simulink model "PMSM_Simulink"  (R2024b)
settings: Solver=FixedStepDiscrete  StartTime=0.0  StopTime=10  FixedStep=0.0000625/200  RelTol=1e-3
libraries: simulink x12, slpidlib x3, spsDCVoltageSourceLib x1, spsPermanentMagnetSynchronousMachineLib x1, spsUniversalBridgeLib x1, sps_lib x1
(part 2 of 2)

== stateflow chart PMSM_Simulink/PMSM_MC1/MC_LowFrqTask /MotModeCtr/Chart ==
  state Calibrate
    state Init
      en:
      MotCtrMode = 0;
    state Calibrate1
      en:
      MotCtrMode=1;
      MotCalThetae=1.046;//60°
    state Calibrate2
      en:
      MotOffsetBuff[0]=Ecode_Cnt-166;
      MotCtrMode=2;
      MotCalThetae=2.093;//120°
    state RngChk
      en:
      MotOffsetBuff[1]=Ecode_Cnt-333;
      RangeCheck();
    (default) -> Init
    Init -> Calibrate1 : [MotorSpdRef !=0]
    Calibrate1 -> Calibrate2 : [after(1.5,sec )]
    Calibrate2 -> RngChk : [after(1.5,sec )]
  state RangeCheck [function]
    (default) -> (junction 31)
    (junction 31) -> (junction 33) [order 1] : [abs(MotOffsetBuff[0]-MotOffsetBuff[1])>1000]
    (junction 33) -> (junction 36) : {
        | MotCalNormal=0;
        | }
    (junction 31) -> (junction 35) [order 2] : {
        | MotCalNormal=1;
        | MotOffset=(MotOffsetBuff[0]+MotOffsetBuff[1]/2)
        | }
    (junction 36) -> (junction 35)
    (junction 35) -> (junction 42)
  state Normal
    state Stop
      en:
      MotCtrMode=4;
    state Run
      en:
      MotCtrMode=5;
    (default) -> Stop
    Run -> Stop : [MotorSpdRef==0]
    Stop -> Run : [MotorSpdRef!=0]
  state CallFailed
    en:
    MotCtrMode=3;
  (default) -> Calibrate
  CallFailed -> Calibrate : [MotorSpdRef==0]
  RngChk -> CallFailed [order 1] : [MotCalNormal==0]
  RngChk -> Normal [order 2] : [MotCalNormal==1]
  data: MotCtrMode output uint8; MotorSpdRef input int16; Ecode_Cnt input int32; MotOffset output int32; MotCalThetae output single; MotOffsetBuff local int32 size=2; MotCalNormal local boolean
